simulink model "ARDroneReplay_V2"  (R2017b)
settings: Solver=ode1  StartTime=0.0  StopTime=30  FixedStep=sampleTime  RelTol=1e-3  EnableMultiTasking=on
undefined symbols (not defined in the file or in its folder): sampleTime
libraries: ARBlocks x2
CloseFcn:
  | rtwprivate ssgencode ModelCloseRequest Good_NL_model
settings Model: ExtModeTrigDuration=100000  Creator=Paul  LastModifiedBy=ritac
settings DataIOCC: LimitDataPoints=on  SaveFormat=Array  SignalLoggingSaveFormat=ModelDataLogs  TimeSaveName=time
settings OptimizationCC: ExpressionDepthLimit=2147483647  InitFltsAndDblsToZero=on
settings DebuggingCC: UnderspecifiedInitializationDetection=Classic  MergeDetectMultiDrivingBlocksExec=none  SolverPrmCheckMsg=warning  FcnCallInpInsideContextMsg=warning  StateNameClashWarn=warning  SFUnexpectedBacktrackingDiag=warning  SFNoUnconditionalDefaultTransitionDiag=warning  SFExecutionAtInitializationDiag=none
settings HardwareCC: ProdBitPerLong=64  ProdHWDeviceType=Intel->x86-64 (Mac OS X)
settings ModelReferenceCC: PropagateSignalLabelsOutOfModel=off
settings RTWCC: SystemTargetFile=sldrt.tlc  TemplateMakefile=sldrt.tmf  Description=Simulink Desktop Real-Time  RTWCompilerOptimization=on
settings CodeAppCC: MaxIdLength=95  StateflowObjectComments=on
settings SimulinkDesktopRealTimeCC: TargetPreCompLibLocation=/Applications/MATLAB_R2017b.app/toolbox/sldrt/lib/maci64  TargetLangStandard=C89/C90 (ANSI)  SupportVariableSizeSignals=off
settings ConfigComp: CovMetricSettings=dw  CovHtmlReporting=on  CovSaveCumulativeToWorkspaceVar=on  CovSaveSingleToWorkspaceVar=on  CovExternalEMLEnable=off

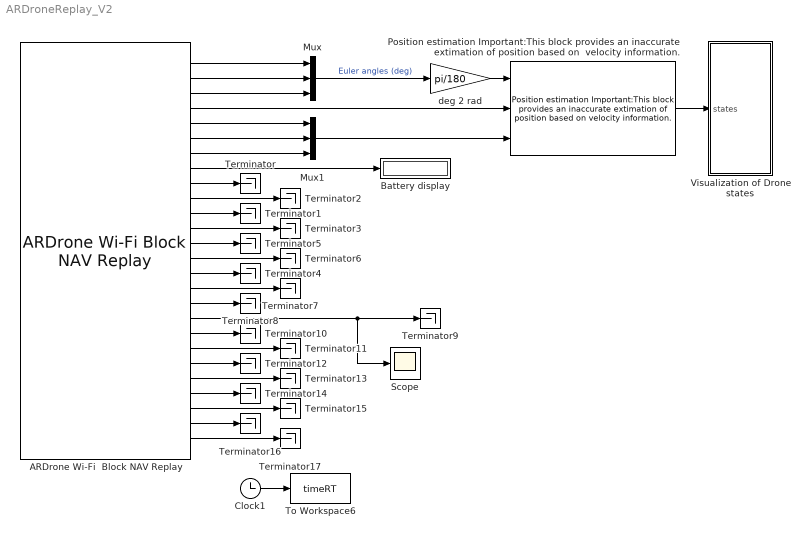
== system ARDroneReplay_V2 ==
  ARDrone Wi-Fi  Block NAV Replay : ARBlocks/ARDrone Wi-Fi  Block NAV Replay
  Battery display : Display
  Clock1 : Clock
  Mux : Mux  Inputs=3
  Mux1 : Mux  Inputs=3
  "Position estimation Important:This block provides an inaccurate extimation of position based on  velocity information. " : ARBlocks/Position estimation Important:This block provides an  inaccurate extimation of position  based on  velocity information. 
  Scope : Scope
  Terminator{,1..17} (18 alike) : Terminator
  To Workspace6 : ToWorkspace  VariableName=timeRT  SampleTime=sampleTime
  Visualization of Drone states : Subsystem
  deg 2 rad : Gain  Gain=pi/180
  wires:
  ARDrone Wi-Fi  Block NAV Replay/1 -> Mux/1
  ARDrone Wi-Fi  Block NAV Replay/2 -> Mux/2
  ARDrone Wi-Fi  Block NAV Replay/5 -> Mux1/1
  ARDrone Wi-Fi  Block NAV Replay/6 -> Mux1/2
  ARDrone Wi-Fi  Block NAV Replay/7 -> Mux1/3
  Mux/1 -> deg 2 rad/1  "Euler angles (deg)"
  ARDrone Wi-Fi  Block NAV Replay/8 -> Battery display/1
  "Position estimation Important:This block provides an inaccurate extimation of position based on  velocity information. "/1 -> Visualization of Drone states/1(states)
  deg 2 rad/1 -> "Position estimation Important:This block provides an inaccurate extimation of position based on  velocity information. "/1
  ARDrone Wi-Fi  Block NAV Replay/4 -> "Position estimation Important:This block provides an inaccurate extimation of position based on  velocity information. "/2
  Mux1/1 -> "Position estimation Important:This block provides an inaccurate extimation of position based on  velocity information. "/3
  ARDrone Wi-Fi  Block NAV Replay/3 -> Mux/3
  ARDrone Wi-Fi  Block NAV Replay/9 -> Terminator/1
  Clock1/1 -> To Workspace6/1
  ARDrone Wi-Fi  Block NAV Replay/15 -> Terminator4/1
  ARDrone Wi-Fi  Block NAV Replay/10 -> Terminator2/1
  ARDrone Wi-Fi  Block NAV Replay/13 -> Terminator5/1
  ARDrone Wi-Fi  Block NAV Replay/14 -> Terminator6/1
  ARDrone Wi-Fi  Block NAV Replay/17 -> Terminator8/1
  ARDrone Wi-Fi  Block NAV Replay/16 -> Terminator7/1
  ARDrone Wi-Fi  Block NAV Replay/19 -> Terminator10/1
  ARDrone Wi-Fi  Block NAV Replay/18 -> Scope/1, Terminator9/1
  ARDrone Wi-Fi  Block NAV Replay/21 -> Terminator12/1
  ARDrone Wi-Fi  Block NAV Replay/20 -> Terminator11/1
  ARDrone Wi-Fi  Block NAV Replay/23 -> Terminator14/1
  ARDrone Wi-Fi  Block NAV Replay/22 -> Terminator13/1
  ARDrone Wi-Fi  Block NAV Replay/25 -> Terminator16/1
  ARDrone Wi-Fi  Block NAV Replay/24 -> Terminator15/1
  ARDrone Wi-Fi  Block NAV Replay/26 -> Terminator17/1
  ARDrone Wi-Fi  Block NAV Replay/11 -> Terminator1/1
  ARDrone Wi-Fi  Block NAV Replay/12 -> Terminator3/1

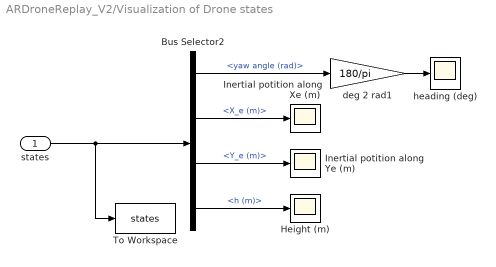
== system ARDroneReplay_V2/Visualization of Drone states ==
  states : Inport
  Bus Selector2 : BusSelector  OutputSignals=yaw angle (rad),X_e (m),Y_e (m),h (m)
  Height (m) : Scope
  Inertial potition along Xe (m) : Scope
  Inertial potition along Ye (m) : Scope
  To Workspace : ToWorkspace  VariableName=states  SaveFormat=Structure With Time  SampleTime=-1
  deg 2 rad1 : Gain  Gain=180/pi
  heading (deg) : Scope
  wires:
  states/1 -> To Workspace/1, Bus Selector2/1
  Bus Selector2/1 -> deg 2 rad1/1  "<yaw angle (rad)>"
  Bus Selector2/2 -> Inertial potition along Xe (m)/1  "<X_e (m)>"
  Bus Selector2/3 -> Inertial potition along Ye (m)/1  "<Y_e (m)>"
  Bus Selector2/4 -> Height (m)/1  "<h (m)>"
  deg 2 rad1/1 -> heading (deg)/1
